simulink model "example1"  (Simulink 7.5)
settings: Solver=FixedStepDiscrete  StartTime=0.0  StopTime=10.0  FixedStep=0.001  RelTol=1e-3
undefined symbols (not defined in the file or in its folder): OC1max
libraries: dsPICdrivers x2
settings Model: Creator=Jose Antoniooooooooo  LastModifiedBy=Jose Antoniooooooooo
settings OptimizationCC: OptimizeModelRefInitCode=on  LifeSpan=1
settings HardwareCC: ProdBitPerInt=16  ProdEndianess=LittleEndian  ProdWordSize=16  ProdHWDeviceType=16-bit Generic
settings RTWCC: SystemTargetFile=dspic.tlc  MakeCommand=make_CreateMPLAB  TemplateMakefile=dspic_pic30_gcc.tmf  PostCodeGenCommand=dsPIC_Compile()  Description=Embedded Target for Microchip dsPIC (real-time)  ProcessScript=dspic_make_rtw_hook
settings CodeAppCC: IgnoreCustomStorageClasses=off
settings STFCustomTargetCC: IncludeMdlTerminateFcn=off  CombineOutputUpdateFcns=on  SuppressErrorStatus=on  ERTCustomFileBanners=on  SupportContinuousTime=off  SupportNonInlinedSFcns=off  SystemTargetFile=dspic.tlc
settings ERTTargetCC: MultiwordLength=2048  ParMdlRefBuildCompliant=off  CompOptLevelCompliant=off  IncludeMdlTerminateFcn=off  SuppressErrorStatus=on  ERTFirstTimeCompliant=off  ModelStepFunctionPrototypeControlCompliant=off  CPPClassGenCompliant=off  InlinedParameterPlacement=NonHierarchical  ERTSrcFileBannerTemplate=dsPIC_code_template.cgt  ERTHdrFileBannerTemplate=dsPIC_code_template.cgt  ERTDataSrcFileTemplate=dsPIC_code_template.cgt  ERTDataHdrFileTemplate=dsPIC_code_template.cgt  ERTCustomFileTemplate=dsPIC_main.tlc  ConvertIfToSwitch=off
settings CustomProperty: DataType=string  Value=C:\PROGRA~1\MATLAB\R2010a\bin\win32\gmake

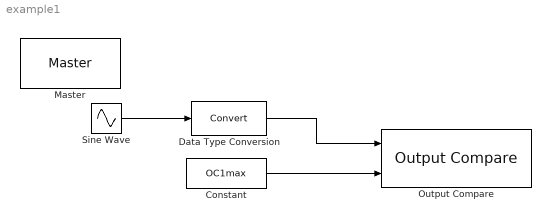
== system example1 ==
  Constant : Constant  Value=OC1max  OutDataTypeMode=uint16  OutDataType=fixdt(1, 16)  OutScaling=2^0  OutDataTypeStr=uint16
  Data Type Conversion : DataTypeConversion  OutDataType=fixdt(1, 16)  OutScaling=2^0
  Master : dsPICdrivers/Master  Tag=dsPIC_MASTER  Priority=1  TimeStepType=Timer1  picType=30f4013  fcy=5e6  Quartz_33f=5e6  PLLActive_33f=off  fcyDesired_33f=0  tmr1="[1  4999  0]"  tmr1Info="Time Step : 0.001  ;   Error : 0%  PR1=4999"  tmr2345="[8  0  0  0]"  tmr2345cfg=[-1 -1 -1 -1]  IOautoConf=on  typePort="[ 0  0  0  0  0  0  0  0  0  0  0  0  0  0  0  0  0  0  0  0  0  0  0  0  0  0  0  0  0  0  0  0  0  0  0  0  0  0  0  0  0  0  0  0  0  0  0  0  7  0  0  0  0  0  0  0  0  0  0  0  0  0  0  0  0  0  0  0  0  0  0  0  0  0  0  0  0  0  0  0  0  0  0  0  0  0  0  0  0  0  0  0  0  0  0  0  0  0  0  0  0  0  0  0  0  0  0  0  0  0  0  0 ]"  TRIS="[ 65535  65535  65535  65534  65535  65535  65535 ]"  ADPCFG=0  MasterBusyPort=None  MasterOverloadPort=None  FOSC=CSW_FSCM_OFF  ClockSwitchMonitor=Both disabled  TempProtection_33f=TEMP_ON  FPBOR=PBOR_OFF  PWRT=PWRT_OFF  MCLR=MCLR_DIS  ICD=ICS_PGD1  JTAGEN=JTAGEN_OFF  PowerSave=off  OverrideFcy=off  NewFcy=1e6  PR2345="[65535  65535  65535  65535]"
  Output Compare : dsPICdrivers/Peripheral I//O/Output Compare  Tag=dsPIC_PWM_out  Priority=5  IntPriority=3  CHANNEL=[1]  Channel_UP_Down_Periode=[5]  MaxChannel=[0.02]  MaxName=' OC1max '  Precision=[13.6094]  Timer=[2]  Status=OK  SafeMarge=[0]  PortLetter=[68]  PortNumber=[0]  MaxValues=[12499]
  Sine Wave : Sin  SineType=Sample based  Amplitude=OC1max/40  Bias=(OC1max/40)*3  Frequency=1  Phase=0  Samples=1000  SampleTime=0.001  Offset=0
  wires:
  Constant/1 -> Output Compare/2
  Data Type Conversion/1 -> Output Compare/1
  Sine Wave/1 -> Data Type Conversion/1
